simulink model "NBMS_DCL"  (R2026b)
settings: Solver=FixedStepDiscrete  StopTime=25
undefined symbols (not defined in the file): VDU_MACHINE_STS_E, X_DCL_30sSAFETY_PACK, X_DCL_CONT_SAFETY_PACK, Y_DCL_30sSAFETY_PACK, Y_DCL_CONT_SAFETY_PACK
libraries: simulink x1
settings Model: Creator=hp  LastModifiedBy=rathi
settings OptimizationCC: DefaultParameterBehavior=Inlined  DifferentSizesBufferReuse=on  EfficientTunableParamExpr=on  EnhancedBackFolding=on  OptimizationCustomize=off  OptimizeBlockOrder=speed  PassReuseOutputArgsAs=Individual arguments  RemoveInternalMemoryZeroInit=on  RemoveRootLevelIOMemoryZeroInit=on
settings DebuggingCC: ParameterTunabilityLossMsg=error
settings SFSimCC: MATLABDynamicMemAlloc=off
settings RTWCC: Description=Embedded Coder  GenCodeOnly=on  PackageGeneratedCodeAndArtifacts=on  SystemTargetFile=ert.tlc  TemplateMakefile=ert_default_tmf
settings CodeAppCC: ForceParamTrailComments=on  IgnoreCustomStorageClasses=off  InsertBlockDesc=on  OperatorAnnotations=on  SFDataObjDesc=on  SimulinkDataObjDesc=on
settings ERTTargetCC: DynamicArrayContainerType=coder::array  GenerateSampleERTMain=on

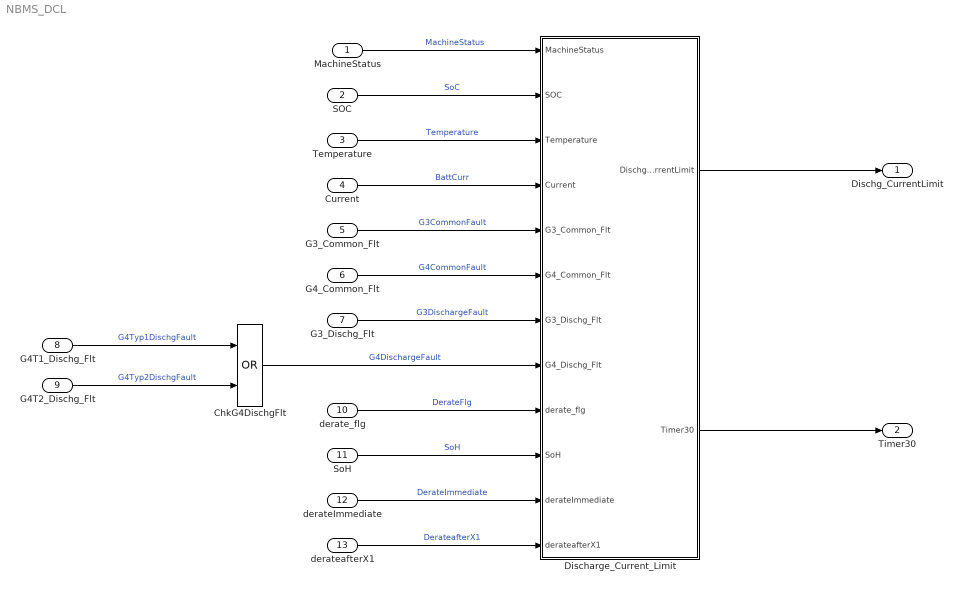
== system NBMS_DCL ==
  MachineStatus : Inport  OutDataTypeStr=Enum: VDU_MACHINE_STS_E
  SOC : Inport  Port=2  OutDataTypeStr=uint8
  Temperature : Inport  Port=3  OutDataTypeStr=double  PortDimensions=[6,1]
  Current : Inport  Port=4
  G3_Common_Flt : Inport  Port=5  OutDataTypeStr=boolean
  G4_Common_Flt : Inport  Port=6  OutDataTypeStr=boolean
  G3_Dischg_Flt : Inport  Port=7  OutDataTypeStr=boolean
  G4T1_Dischg_Flt : Inport  Port=8  OutDataTypeStr=boolean
  G4T2_Dischg_Flt : Inport  Port=9  OutDataTypeStr=boolean
  derate_flg : Inport  Port=10  OutDataTypeStr=boolean
  SoH : Inport  Port=11
  derateImmediate : Inport  Port=12  OutDataTypeStr=boolean
  derateafterX1 : Inport  Port=13  OutDataTypeStr=boolean
  ChkG4DischgFlt : Logic  Operator=OR  AllPortsSameDT=off  OutDataTypeStr=boolean
  Discharge_Current_Limit : Subsystem
  Dischg_CurrentLimit : Outport  OutDataTypeStr=double
  Timer30 : Outport  Port=2  OutDataTypeStr=double
  wires:
  MachineStatus/1 -> Discharge_Current_Limit/1(MachineStatus)  "MachineStatus"
  Temperature/1 -> Discharge_Current_Limit/3(Temperature)  "Temperature"
  SOC/1 -> Discharge_Current_Limit/2(SOC)  "SoC"
  Current/1 -> Discharge_Current_Limit/4(Current)  "BattCurr"
  Discharge_Current_Limit/1(Dischg_CurrentLimit) -> Dischg_CurrentLimit/1
  Discharge_Current_Limit/2(Timer30) -> Timer30/1
  G3_Common_Flt/1 -> Discharge_Current_Limit/5(G3_Common_Flt)  "G3CommonFault"
  G4_Common_Flt/1 -> Discharge_Current_Limit/6(G4_Common_Flt)  "G4CommonFault"
  G3_Dischg_Flt/1 -> Discharge_Current_Limit/7(G3_Dischg_Flt)  "G3DischargeFault"
  ChkG4DischgFlt/1 -> Discharge_Current_Limit/8(G4_Dischg_Flt)  "G4DischargeFault"
  G4T1_Dischg_Flt/1 -> ChkG4DischgFlt/1  "G4Typ1DischgFault"
  G4T2_Dischg_Flt/1 -> ChkG4DischgFlt/2  "G4Typ2DischgFault"
  derate_flg/1 -> Discharge_Current_Limit/9(derate_flg)  "DerateFlg"
  SoH/1 -> Discharge_Current_Limit/10(SoH)  "SoH"
  derateImmediate/1 -> Discharge_Current_Limit/11(derateImmediate)  "DerateImmediate"
  derateafterX1/1 -> Discharge_Current_Limit/12(derateafterX1)  "DerateafterX1"

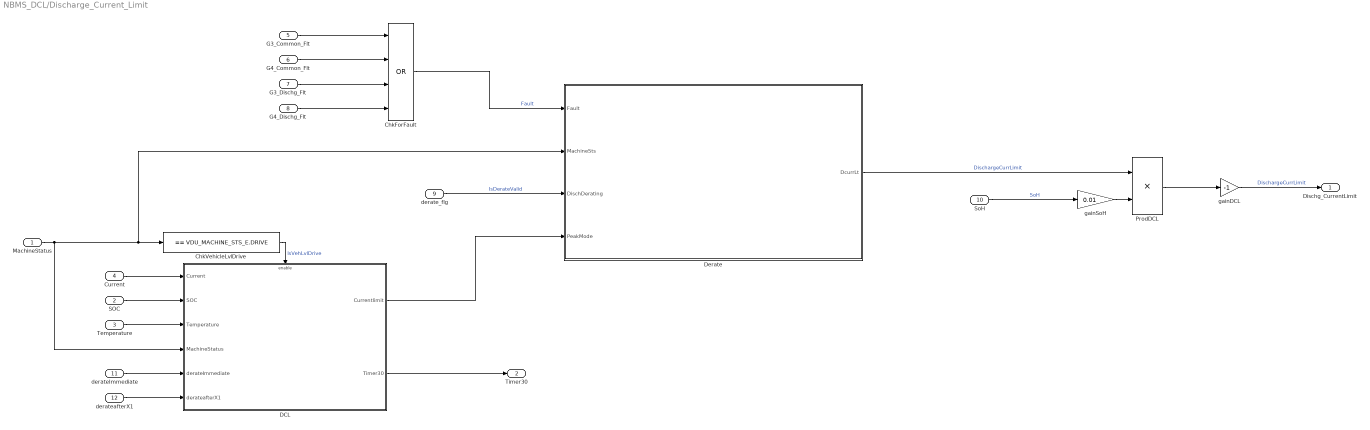
== system NBMS_DCL/Discharge_Current_Limit ==
  MachineStatus : Inport  OutDataTypeStr=Enum: VDU_MACHINE_STS_E
  SOC : Inport  Port=2  OutDataTypeStr=uint8
  Temperature : Inport  Port=3  OutDataTypeStr=double  PortDimensions=[6,1]
  Current : Inport  Port=4
  G3_Common_Flt : Inport  Port=5  OutDataTypeStr=boolean
  G4_Common_Flt : Inport  Port=6  OutDataTypeStr=boolean
  G3_Dischg_Flt : Inport  Port=7  OutDataTypeStr=boolean
  G4_Dischg_Flt : Inport  Port=8  OutDataTypeStr=boolean
  derate_flg : Inport  Port=9
  SoH : Inport  Port=10
  derateImmediate : Inport  Port=11
  derateafterX1 : Inport  Port=12
  ChkForFault : Logic  Operator=OR  Inputs=4  AllPortsSameDT=off  OutDataTypeStr=boolean
  ChkVehicleLvlDrive : simulink/Logic and Bit Operations/Compare To Constant  relop===  const=VDU_MACHINE_STS_E.DRIVE  OutDataTypeStr=boolean
  DCL : Subsystem  TreatAsAtomicUnit=on
  Derate : Stateflow chart  TreatAsAtomicUnit=on
      settings: PortSchema="{\"entries\":[{\"content\":{\"sides\":[{\"content\":{\"connectorIds\":[\"In3\",\"In2\",\"In4\",\"In1\"]},\"type\":\"ConnectorPlacement.EquallySpacedRectSide\",\"uuid\":\"6af2e017-3178-4203-8b2c-26e58e1fbb9e\"},{\"content\":{\"connectorIds\":[\"Out1\"],\"side\":\"RIGHT\"},\"type\":\"ConnectorPlacement.EquallySpacedRectSide\",\"uuid\":\"8c3377ca-a378-4f45-9950-e803323a87dc\"},{\"content\":{\"side\":\"TOP\"},\"type\":\"ConnectorPlacement.EquallySpacedRectSide\",\"uuid\":\"ffab1a59-9d08-45f8-8a9b-e5714e1d35f1\"}]},\"type\":\"ConnectorPlacement.EquallySpacedConnector\",\"uuid\":\"90544a8f-2548-41f0-8509-502794987d44\"}],\"packageUris\":[\"http://schema.mathworks.com/mf0/Connector/R2020b\"],\"version\":\"1.0\"}"
  ProdDCL : Product
  gainDCL : Gain  Gain=-1
  gainSoH : Gain  Gain=0.01
  Dischg_CurrentLimit : Outport  OutDataTypeStr=double
  Timer30 : Outport  Port=2  OutDataTypeStr=double
  wires:
  MachineStatus/1 -> DCL/4(MachineStatus), Derate/2(MachineSts), ChkVehicleLvlDrive/1
  SOC/1 -> DCL/2(SOC)
  Temperature/1 -> DCL/3(Temperature)
  Current/1 -> DCL/1(Current)
  ChkVehicleLvlDrive/1 -> DCL/Enable  "IsVehLvlDrive"
  DCL/2(Timer30) -> Timer30/1
  G4_Common_Flt/1 -> ChkForFault/2
  G3_Common_Flt/1 -> ChkForFault/1
  G3_Dischg_Flt/1 -> ChkForFault/3
  G4_Dischg_Flt/1 -> ChkForFault/4
  ChkForFault/1 -> Derate/3(Fault)  "Fault"
  DCL/1(Currentlimit) -> Derate/1(PeakMode)
  derate_flg/1 -> Derate/4(DischDerating)  "IsDerateValid"
  Derate/1(DcurrLt) -> ProdDCL/1  "DischargeCurrLimit"
  SoH/1 -> gainSoH/1  "SoH"
  gainSoH/1 -> ProdDCL/2
  ProdDCL/1 -> gainDCL/1
  gainDCL/1 -> Dischg_CurrentLimit/1  "DischargeCurrLimit"
  derateImmediate/1 -> DCL/5(derateImmediate)
  derateafterX1/1 -> DCL/6(derateafterX1)

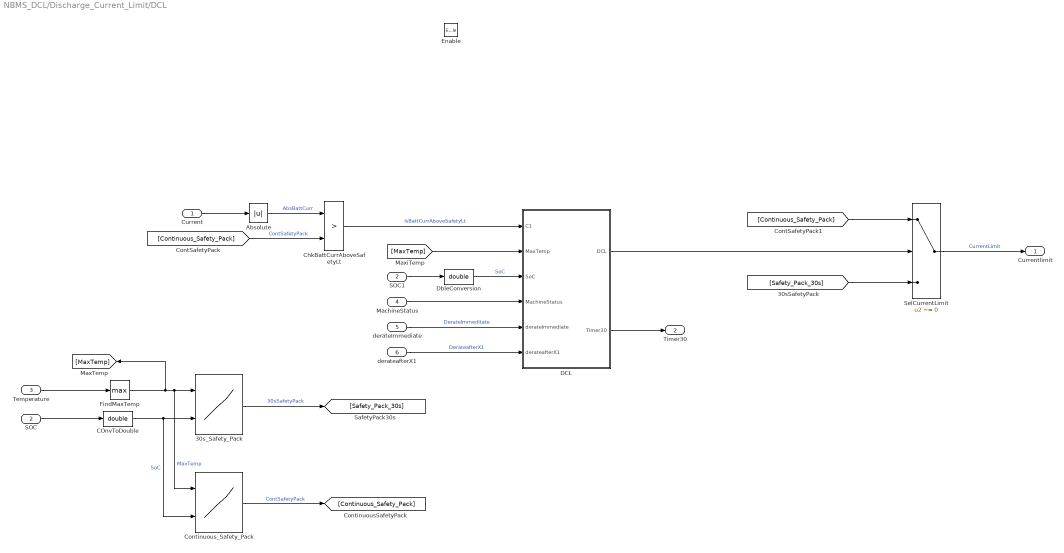
== system NBMS_DCL/Discharge_Current_Limit/DCL ==
  Current : Inport
  SOC : Inport  Port=2  OutDataTypeStr=uint8
  Temperature : Inport  Port=3  OutDataTypeStr=double  PortDimensions=[6,1]
  MachineStatus : Inport  Port=4  OutDataTypeStr=Enum: VDU_MACHINE_STS_E
  derateImmediate : Inport  Port=5  OutDataTypeStr=boolean
  derateafterX1 : Inport  Port=6
  Enable : EnablePort  StatesWhenEnabling=reset
  30s_Safety_Pack : Lookup_n-D  BreakpointsForDimension1=X_DCL_30sSAFETY_PACK  BreakpointsForDimension2=Y_DCL_30sSAFETY_PACK  Table=[0 0 0 0 0 0 0 0 0 0 0 0 0;0 0 0 0 0 0 0 0 0 0 0 0 0;0 7 14 56 77 91 98 105 110 110 110 110 110;14 14 35 84 110 110 110 110 110 110 110 110 110;20 21 56 110 110 110 110 110 110 110 110 110 110;20 42 84 110 110 110 110 110 110 110 110 110 110;20 42 84 110 110 110 110 110 110 110 110 110 110;20 42 84 110 110 110 110 110 110 110 110 110 110;20 35 52 98 110 110 110 110 110 110 110 110 110;0 0 0 0 0 0 0 0 0 0 0 0 0]  InternalRulePriority=Speed  RndMeth=Simplest
      settings: InputPortMap=u0,u1
  Absolute : Abs  SaturateOnIntegerOverflow=off
  COnvToDouble : DataTypeConversion  OutDataTypeStr=double  SaturateOnIntegerOverflow=off  RndMeth=Floor
  ChkBattCurrAboveSafetyLt : RelationalOperator  Operator=>  OutDataTypeStr=boolean  RndMeth=Simplest  InputSameDT=off
  Continuous_Safety_Pack : Lookup_n-D  BreakpointsForDimension1=X_DCL_CONT_SAFETY_PACK  BreakpointsForDimension2=Y_DCL_CONT_SAFETY_PACK  Table=[0 0 0 0 0 0 0 0 0 0 0 0 0;0 0 0 0 0 0 0 0 0 0 0 0 0;0 7 14 21 21 31 31 31 31 31 31 31 31;14 14 35 52 52 52 52 52 52 52 52 52 52;20 21 56 70 84 84 84 84 84 84 84 84 84;20 42 42 70 90 90 90 90 90 90 90 90 90;20 42 42 70 90 90 90 90 90 90 90 90 90;20 42 42 52.5 90 90 90 90 90 90 90 90 90;20 28 35 35 35 35 35 35 35 35 35 35 35;0 0 0 0 0 0 0 0 0 0 0 0 0;]  InternalRulePriority=Speed  RndMeth=Simplest
      settings: InputPortMap=u0,u1
  DCL : Subsystem
  DbleConversion : DataTypeConversion  OutDataTypeStr=double  SaturateOnIntegerOverflow=off  RndMeth=Floor
  FindMaxTemp : MinMax  Function=max
  SOC1 : InportShadow  Port=2  OutDataTypeStr=uint8
  SelCurrentLimit : Switch  Criteria=u2 ~= 0  SaturateOnIntegerOverflow=off  InputSameDT=off
  Currentlimit : Outport  OutputWhenDisabled=reset  InitialOutput=0
  Timer30 : Outport  Port=2
  wires:
  Current/1 -> Absolute/1
  Absolute/1 -> ChkBattCurrAboveSafetyLt/1  "AbsBattCurr"
  Temperature/1 -> FindMaxTemp/1
  SOC/1 -> COnvToDouble/1
  FindMaxTemp/1 -> [MaxTemp], Continuous_Safety_Pack/1, 30s_Safety_Pack/1  "MaxTemp"
  COnvToDouble/1 -> Continuous_Safety_Pack/2, 30s_Safety_Pack/2  "SoC"
  30s_Safety_Pack/1 -> [Safety_Pack_30s]  "30sSafetyPack"
  Continuous_Safety_Pack/1 -> [Continuous_Safety_Pack]  "ContSafetyPack"
  [Continuous_Safety_Pack] -> ChkBattCurrAboveSafetyLt/2  "ContSafetyPack"
  [Continuous_Safety_Pack] -> SelCurrentLimit/1
  [Safety_Pack_30s] -> SelCurrentLimit/3
  SelCurrentLimit/1 -> Currentlimit/1  "CurrentLimit"
  ChkBattCurrAboveSafetyLt/1 -> DCL/1(C1)  "IsBattCurrAboveSafetyLt"
  DCL/2(Timer30) -> Timer30/1
  DCL/1(DCL) -> SelCurrentLimit/2
  [MaxTemp] -> DCL/2(MaxTemp)
  SOC1/1 -> DbleConversion/1
  MachineStatus/1 -> DCL/4(MachineStatus)
  DbleConversion/1 -> DCL/3(SoC)  "SoC"
  derateImmediate/1 -> DCL/5(derateImmediate)  "DerateImmeditate"
  derateafterX1/1 -> DCL/6(derateafterX1)  "DerateafterX1"

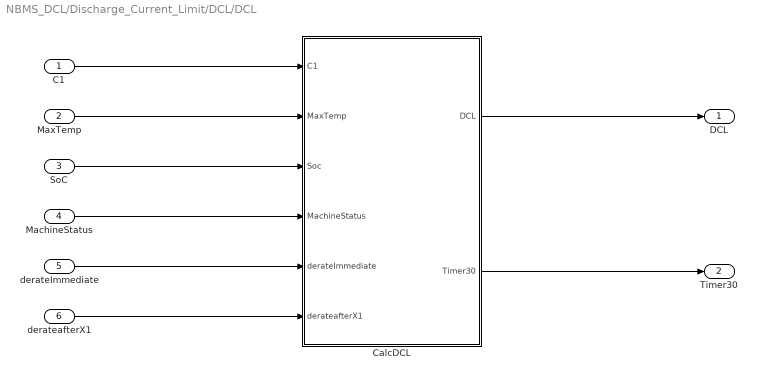
== system NBMS_DCL/Discharge_Current_Limit/DCL/DCL ==
  C1 : Inport
  MaxTemp : Inport  Port=2
  SoC : Inport  Port=3
  MachineStatus : Inport  Port=4  OutDataTypeStr=Enum: VDU_MACHINE_STS_E
  derateImmediate : Inport  Port=5  OutDataTypeStr=boolean
  derateafterX1 : Inport  Port=6  OutDataTypeStr=boolean
  CalcDCL : Stateflow chart  TreatAsAtomicUnit=on
  DCL : Outport
  Timer30 : Outport  Port=2
  wires:
  CalcDCL/2(Timer30) -> Timer30/1
  MaxTemp/1 -> CalcDCL/2(MaxTemp)
  C1/1 -> CalcDCL/1(C1)
  SoC/1 -> CalcDCL/3(Soc)
  MachineStatus/1 -> CalcDCL/4(MachineStatus)
  CalcDCL/1(DCL) -> DCL/1
  derateImmediate/1 -> CalcDCL/5(derateImmediate)
  derateafterX1/1 -> CalcDCL/6(derateafterX1)

== stateflow chart NBMS_DCL/Discharge_Current_Limit/DCL/DCL/CalcDCL ==
  state Continuous
    en,du:
    DCL = 1;
  state C1_Condition
    state Peak
      en,du:
      if (Timer30>0)
      Timer30 = Timer30 - 0.1;
      end
    state C1_Advantage
      en,du:
      if (Timer30<30)
      Timer30 = Timer30 + 0.1
      end
    (default) -> (junction 5) : {Timer30 = 30;
        | DCL = 0;}
    (junction 5) -> (junction 9) [order 1] : [C1 == 0]
    (junction 5) -> Peak [order 2]
    (junction 9) -> C1_Advantage
    Peak -> C1_Advantage : [C1 == 0]
    C1_Advantage -> Peak : [C1 == 1]
  (default) -> (junction 26)
  Continuous -> (junction 26) [order 1] : [MachineStatus ~= VDU_MACHINE_STS_E.DRIVE]
  (junction 26) -> Continuous [order 2]
  (junction 26) -> C1_Condition [order 1] : [(Soc > 20) && (MaxTemp<=47 && MaxTemp >=10)]
  C1_Condition -> Continuous [order 1] : [Timer30 <= 0]
  C1_Condition -> Continuous [order 2] : [(duration(derateafterX1 == true) >=10) || derateImmediate==true || MaxTemp>=47 || MaxTemp <10]
  Continuous -> C1_Condition [order 2] : [derateafterX1==false && derateImmediate==false && (MaxTemp<=47 && MaxTemp >=10)]
  data: DCL output; C1 input; Timer30 output; MaxTemp input; Soc input; MachineStatus input; derateImmediate input; derateafterX1 input

== stateflow chart NBMS_DCL/Discharge_Current_Limit/Derate ==
  state IDLE
    DcurrLt = 0;
  state DRIVE
    state G2_Derating
      state G2_min
        en,du:
        DcurrLt = PeakMode;
        time=elapsed(sec);
      state G2_Eco
        DcurrLt= min(60,PeakMode);
      (default) -> G2_min
      G2_min -> G2_Eco : [time>=10]
    state PeakMode
      en,du:
      DcurrLt = PeakMode;
    (default) -> PeakMode
    PeakMode -> G2_Derating : [DischDerating == true]
    G2_Derating -> PeakMode : [DischDerating == false]
  (default) -> IDLE
  IDLE -> DRIVE : [MachineSts == VDU_MACHINE_STS_E.DRIVE && ...
      | Fault == false]
  DRIVE -> IDLE : [MachineSts ~= VDU_MACHINE_STS_E.DRIVE || ...
      | Fault == true]
  data: DcurrLt output; time local; PeakMode input; MachineSts input; Fault input; DischDerating input
